simulink model "Pack_Lumped"  (R2026b)
settings: Solver=VariableStepAuto
undefined symbols (not defined in the file or in its folder): P, Ts
libraries: Shaddad_Battery_Lumped_lib x1
settings Model: Creator=aomar  LastModifiedBy=aomar

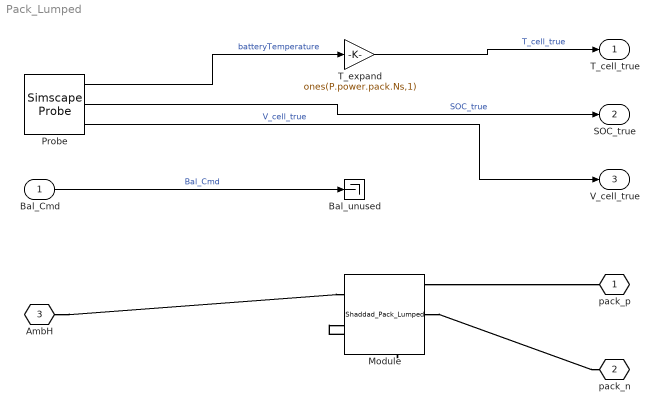
== system Pack_Lumped ==
  Bal_Cmd : Inport  OutDataTypeStr=boolean  PortDimensions=P.power.pack.Ns  SampleTime=Ts.bms_fast
  Bal_unused : Terminator
  Module : Shaddad_Battery_Lumped_lib/Shaddad_Pack_Lumped  BatteryCapacityCell=P.power.cell.Q_Ah*P.power.pack.age.cap_factor A*hr  ExtrapolationMethodCell=simscape.enum.extrapolation.linear  SOCBreakpointsCell=P.power.cell.SOC_bp  TemperatureBreakpointsCell=P.power.cell.T_bp K  OpenCircuitVoltageThermalCell=P.power.cell.OCV_tab V  VoltageRangeCell=P.power.cell.VoltageRange V  ResistanceSOCBreakpointsCell=P.power.cell.SOC_bp  ResistanceTemperatureBreakpointsCell=P.power.cell.T_bp K  R0ThermalCell=P.power.cell.R0_tab*P.power.pack.age.R0_factor Ohm  R1ThermalCell=P.power.cell.R1_tab Ohm  Tau1ThermalCell=P.power.cell.tau1_tab s  BatteryThermalMassCell=P.power.cell.Cth J/K  AmbientResistance=P.power.pack.R_amb_cell K/W  NonCellElectricalResistance=P.power.pack.R_noncell_total Ohm  socCell_specify=on  socCell_priority=High  socCell=mean(P.power.pack.var.SOC0_vec)  socCell_nominal_specify=off  socCell_nominal_value=1  socCell_nominal_unit=1  batteryVoltage_specify=off  batteryVoltage_priority=None  batteryVoltage=0 V  batteryVoltage_nominal_specify=off  batteryVoltage_nominal_value=1  batteryVoltage_nominal_unit=V  batteryCurrent_specify=off  batteryCurrent_priority=None  batteryCurrent=0 A  batteryCurrent_nominal_specify=off  batteryCurrent_nominal_value=1  batteryCurrent_nominal_unit=A  numCycles_specify=off  numCycles_priority=High  numCycles=0  numCycles_nominal_specify=off  numCycles_nominal_value=1  numCycles_nominal_unit=1  batteryTemperature_specify=on  batteryTemperature_priority=High  batteryTemperature=P.power.thermal.T_init_K K  batteryTemperature_nominal_specify=off  batteryTemperature_nominal_value=1  batteryTemperature_nominal_unit=K  vParallelAssembly_specify=off  vParallelAssembly_priority=None  vParallelAssembly=repmat(0, 13, 1) V  vParallelAssembly_nominal_specify=off  vParallelAssembly_nominal_value=1  vParallelAssembly_nominal_unit=V  socParallelAssembly_specify=off  socParallelAssembly_priority=None  socParallelAssembly=repmat(1, 13, 1)  socParallelAssembly_nominal_specify=off  socParallelAssembly_nominal_value=1  socParallelAssembly_nominal_unit=1
  Probe : SimscapeProbe  BoundBlock=8  Variables="{\"batteryTemperature\":{\"Probing\":\"ON\"},\"socParallelAssembly\":{\"Probing\":\"ON\"},\"vParallelAssembly\":{\"Probing\":\"ON\"}}"
  T_expand : Gain  Gain=ones(P.power.pack.Ns,1)
  pack_p : PMIOPort  Side=Right  ConnectionType=Connection: foundation.electrical.electrical
  pack_n : PMIOPort  Port=2  Side=Right  ConnectionType=Connection: foundation.electrical.electrical
  AmbH : PMIOPort  Port=3  Side=Left  ConnectionType=Connection: foundation.thermal.thermal
  T_cell_true : Outport  OutDataTypeStr=double
  SOC_true : Outport  Port=2  OutDataTypeStr=double
  V_cell_true : Outport  Port=3  OutDataTypeStr=double
  wires:
  Bal_Cmd/1 -> Bal_unused/1  "Bal_Cmd"
  Probe/1 -> T_expand/1  "batteryTemperature"
  Probe/2 -> SOC_true/1  "SOC_true"
  Probe/3 -> V_cell_true/1  "V_cell_true"
  T_expand/1 -> T_cell_true/1  "T_cell_true"
  connections:
  AmbH/RConn1 -- Module/LConn1
  Module/LConn2 -- pack_p/RConn1
  Module/RConn1 -- pack_n/RConn1
